simulink model "RNN_simulation_comparaison"  (R2026b)
settings: Solver=VariableStepAuto  StopTime=100*Ts
values from neighbouring files (symbols this model uses):
  bf = evalin('base','bf')    [EKF_MeasurementFcn_coder_ext.m]
  bxu = evalin('base','bxu')    [EKF_StateTransitionFcn_coder_ext.m]
  coef_input = evalin('base','coef_input')    [EKF_StateTransitionFcn_coder_ext.m]
  T0 = evalin('base','T0')    [EKF_MeasurementFcn_coder_ext.m]
  Ts = 0.05    [random_init.m]
  Wf = evalin('base','Wf')    [EKF_MeasurementFcn_coder_ext.m]
  Wu = evalin('base','Wu')    [EKF_StateTransitionFcn_coder_ext.m]
  Wx = evalin('base','Wx')    [EKF_StateTransitionFcn_coder_ext.m]
  y_span = evalin('base','y_span')    [EKF_MeasurementFcn_coder_ext.m]
undefined symbols (not defined in the file or in its folder): A, Cth, emissivity, h, nx, Ta
settings Model: Creator=chalqua  LastModifiedBy=chalqua

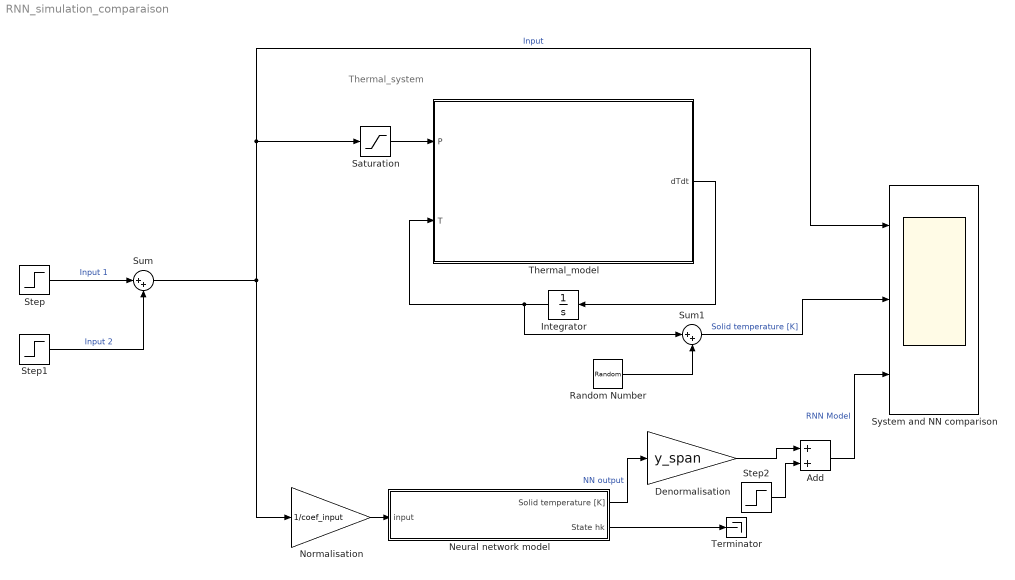
== system RNN_simulation_comparaison ==
  note: Thermal_system
  Add : Sum
  Denormalisation : Gain  Gain=y_span
  Integrator : Integrator  InitialCondition=T0
  Neural network model : Subsystem
  Normalisation : Gain  Gain=1/coef_input
  Random Number : RandomNumber  Variance=0.02  Seed=84198  SampleTime=190
  Saturation : Saturate  UpperLimit=20  LowerLimit=-20
  Step : Step  Time=10*Ts  FinalValue=5  SampleTime=0
  Step1 : Step  Time=40*Ts  FinalValue=-17  SampleTime=0
  Step2 : Step  Time=0  InitialValue=T0  FinalValue=T0  SampleTime=0
  Sum : Sum  Inputs=|++
  Sum1 : Sum  Inputs=|++
  System and NN comparison : Scope  NumInputPorts=3
      settings: ActiveDisplayYMinimum=-18.511633782040342  ActiveDisplayYMaximum=15.326823731573262
  Terminator : Terminator
  Thermal_model : MATLAB Function  TreatAsAtomicUnit=on
  wires:
  Neural network model/1(Solid temperature [K]) -> Denormalisation/1  "NN output"
  Normalisation/1 -> Neural network model/1(input)
  Sum1/1 -> System and NN comparison/2  "Solid temperature [K]"
  Integrator/1 -> Sum1/1, Thermal_model/2(T)
  Add/1 -> System and NN comparison/3  "RNN Model"
  Step/1 -> Sum/1  "Input 1"
  Denormalisation/1 -> Add/1
  Neural network model/2(State hk) -> Terminator/1
  Step1/1 -> Sum/2  "Input 2"
  Thermal_model/1(dTdt) -> Integrator/1
  Random Number/1 -> Sum1/2
  Step2/1 -> Add/2
  Saturation/1 -> Thermal_model/1(P)
  Sum/1 -> Normalisation/1, Saturation/1, System and NN comparison/1  "Input"

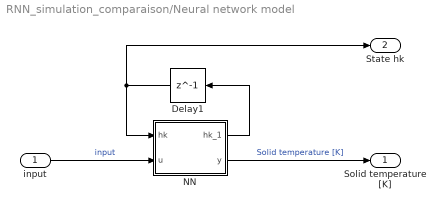
== system RNN_simulation_comparaison/Neural network model ==
  input : Inport
  Delay1 : Delay  DelayLength=1  InitialCondition=zeros(nx,1)  SampleTime=Ts
  NN : MATLAB Function  TreatAsAtomicUnit=on  SystemSampleTime=Ts
  Solid temperature [K] : Outport
  State hk : Outport  Port=2
  wires:
  Delay1/1 -> NN/1(hk), State hk/1
  NN/1(hk_1) -> Delay1/1
  input/1 -> NN/2(u)  "input"
  NN/2(y) -> Solid temperature [K]/1  "Solid temperature [K]"

== matlab function RNN_simulation_comparaison/Neural network model/NN ==
  data: hk input; u input; hk_1 output; y output; Wx parameter; Wf parameter; bxu parameter; bf parameter; Wu parameter
function [hk_1,y] = fcn(hk,u,Wx, Wf, bxu, bf, Wu)

    % Wrapper function for the neural network submarine model
    % Calls the 'thermal_model_NN' function to update hidden state and output
    % Inputs:
    %   hk  - current hidden state vector
    %   u   - control input
    %   Wx  - hidden-to-hidden weight matrix
    %   Wf  - hidden-to-output weight vector
    %   bxu - hidden layer bias vector
    %   bf  - output layer bias
    %   Wu  - input-to-hidden weight vector
    % Outputs:
    %   hk_1 - updated hidden state at next time step
    %   y    - output of the neural network

    [hk_1,y] = thermal_model_NN(hk,u,Wx, Wf, bxu, bf, Wu);
    
end

== matlab function RNN_simulation_comparaison/Thermal_model ==
  data: P input; dTdt output; T input; emissivity parameter; Ta parameter; A parameter; h parameter; Cth parameter
function dTdt = thermal_model(P, T, emissivity, Ta, A, h, Cth)
    %#codegen
    % Continuous-time nonlinear thermal model.
    %
    % Inputs:
    %   P          - Heating power [W]
    %   T          - Solid temperature [K]
    %   Cth        - Thermal capacitance [J/K]
    %   h          - Convective heat transfer coefficient [W/(m^2 K)]
    %   A          - Heat exchange surface area [m^2]
    %   emissivity - Surface emissivity [-]
    %   Ta         - Ambient temperature [K]
    %
    % Output:
    %   dTdt       - Temperature derivative [K/s]
    %
    % Model assumptions:
    %   - Uniform temperature inside the solid
    %   - Constant ambient temperature
    %   - Constant physical parameters
    
    % Stefan-Boltzmann constant [W/(m^2 K^4)]
    sigma = 5.670374419e-8;
    
    % Convective heat losses [W]
    Qconv = h * A * (T - Ta);
    
    % Radiative heat losses [W]
    Qrad = emissivity * sigma * A * (T^4 - Ta^4);
    
    % Compute the temperature derivative [K/s]
    dTdt = (P - Qconv - Qrad) / Cth;

end
